simulink model "test_twin1d"  (R2024b)
settings: Solver=FixedStepDiscrete  StartTime=0.0  StopTime=8  FixedStep=2e-4  RelTol=1e-3
undefined symbols (not defined in the file): S_abdominal, S_lower, S_upper
settings Model: Creator=sammy  LastModifiedBy=sammy

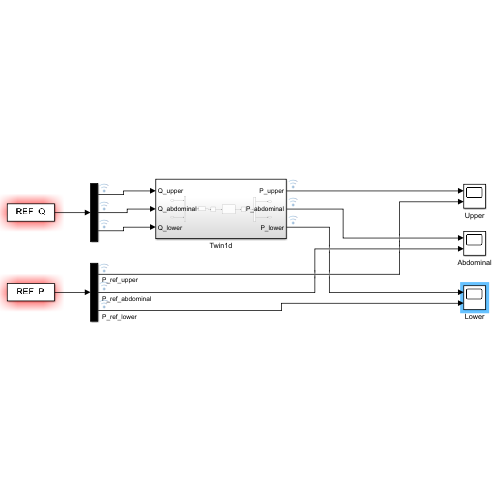
[thumbnail: Simulink's stored preview of the top-level diagram]
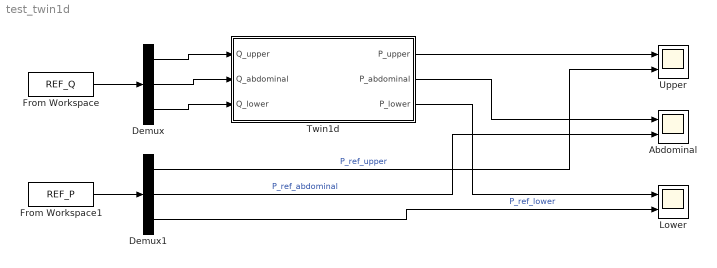
== system test_twin1d ==
  Abdominal : Scope  NumInputPorts=2
  Demux : Demux  Outputs=3
  Demux1 : Demux  Outputs=3
  From Workspace : FromWorkspace  VariableName=REF_Q  SampleTime=2e-4
  From Workspace1 : FromWorkspace  VariableName=REF_P  SampleTime=2e-4
  Lower : Scope  NumInputPorts=2
  Twin1d : Subsystem
  Upper : Scope  NumInputPorts=2
  wires:
  From Workspace/1 -> Demux/1
  Demux/3 -> Twin1d/3(Q_lower)
  Demux/2 -> Twin1d/2(Q_abdominal)
  Demux/1 -> Twin1d/1(Q_upper)
  From Workspace1/1 -> Demux1/1
  Demux1/1 -> Upper/2  "P_ref_upper"
  Twin1d/1(P_upper) -> Upper/1
  Demux1/2 -> Abdominal/2  "P_ref_abdominal"
  Twin1d/2(P_abdominal) -> Abdominal/1
  Twin1d/3(P_lower) -> Lower/1
  Demux1/3 -> Lower/2  "P_ref_lower"

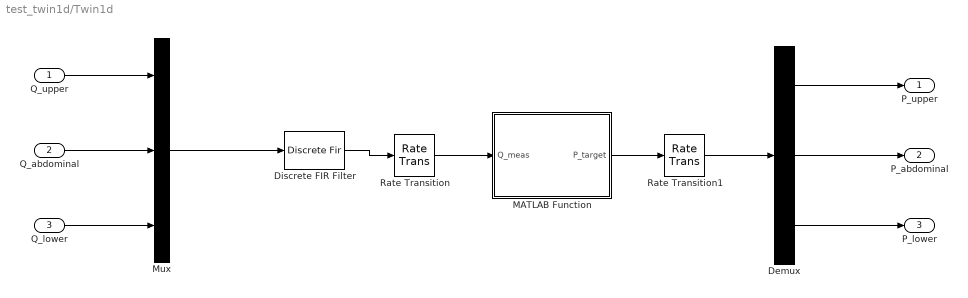
== system test_twin1d/Twin1d ==
  Q_upper : Inport
  Q_abdominal : Inport  Port=2
  Q_lower : Inport  Port=3
  Demux : Demux  Outputs=3
  Discrete FIR Filter : DiscreteFir  Coefficients=ones(1,5)/5
  MATLAB Function : MATLAB Function  TreatAsAtomicUnit=on
  Mux : Mux  Inputs=3
  Rate Transition : RateTransition  OutPortSampleTime=1e-3
  Rate Transition1 : RateTransition  OutPortSampleTime=2e-4
  P_upper : Outport
  P_abdominal : Outport  Port=2
  P_lower : Outport  Port=3
  wires:
  Q_upper/1 -> Mux/1
  Q_abdominal/1 -> Mux/2
  Q_lower/1 -> Mux/3
  Mux/1 -> Discrete FIR Filter/1
  Discrete FIR Filter/1 -> Rate Transition/1
  Rate Transition/1 -> MATLAB Function/1(Q_meas)
  MATLAB Function/1(P_target) -> Rate Transition1/1
  Rate Transition1/1 -> Demux/1
  Demux/1 -> P_upper/1
  Demux/2 -> P_abdominal/1
  Demux/3 -> P_lower/1

== matlab function test_twin1d/Twin1d/MATLAB Function ==
  data: Q_meas input; P_target output; S_upper parameter; S_abdominal parameter; S_lower parameter
function P_target = twin_chambers_block(Q_meas, S_upper, S_abdominal, S_lower)
%TWIN_CHAMBERS_BLOCK  Body of the MATLAB Function block "Twin1D".
%   One block for the three Windkessel chambers.
%   Q_meas   [mL/s] 3x1 flow measured INTO each chamber (positive entering):
%                   [upper; abdominal; lower]
%   S_upper, S_abdominal, S_lower: 1D sub-trees from parameters_chamber1d.m,
%                   NON-TUNABLE parameters of the block
%   P_target [mmHg] 3x1 pressure each chamber must reproduce
%   Block sample time 1e-3 s (= S_*.dt), one solver step per call.
%#codegen
persistent Au Qu Pnu Pcu  Aa Qa Pna Pca  Al Ql Pnl Pcl
if isempty(Au)                                  % rest at P = DBP
    Au = S_upper.A0;      Qu = zeros(S_upper.nF,1);
    Pnu = S_upper.Pref*ones(S_upper.nNodes,1);      Pcu = S_upper.Pref*ones(numel(S_upper.tSeg),1);
    Aa = S_abdominal.A0;  Qa = zeros(S_abdominal.nF,1);
    Pna = S_abdominal.Pref*ones(S_abdominal.nNodes,1); Pca = S_abdominal.Pref*ones(numel(S_abdominal.tSeg),1);
    Al = S_lower.A0;      Ql = zeros(S_lower.nF,1);
    Pnl = S_lower.Pref*ones(S_lower.nNodes,1);      Pcl = S_lower.Pref*ones(numel(S_lower.tSeg),1);
end
[Au, Qu, Pnu, Pcu] = charlton1d_step(S_upper,     Au, Qu, Pnu, Pcu, 1e-6*Q_meas(1));
[Aa, Qa, Pna, Pca] = charlton1d_step(S_abdominal, Aa, Qa, Pna, Pca, 1e-6*Q_meas(2));
[Al, Ql, Pnl, Pcl] = charlton1d_step(S_lower,     Al, Ql, Pnl, Pcl, 1e-6*Q_meas(3));
P_target = [Pnu(S_upper.root); Pna(S_abdominal.root); Pnl(S_lower.root)]/133.322;
end
